simulink model "TP_Lab2_PI_TL081"  (R2026b)
settings: Solver=ode23t  StopTime=0.08  MaxStep=1e-5  RelTol=1e-6  AbsTol=1e-8
libraries: fl_lib x28, ee_lib x5, nesl_utility x3
settings Model: Creator=Usuario  LastModifiedBy=Usuario
settings SimscapeCC: SimscapeLogType=all  SimscapeNominalValues="[{\"value\":\"1\",\"unit\":\"A\"},{\"value\":\"1\",\"unit\":\"bar\"},{\"value\":\"1\",\"unit\":\"cm^2\"},{\"value\":\"1\",\"unit\":\"cm^3/s\"},{\"value\":\"1\",\"unit\":\"kJ/kg\"},{\"value\":\"1\",\"unit\":\"kW\"},{\"value\":\"1\",\"unit\":\"l\"},{\"value\":\"1\",\"unit\":\"N\"},{\"value\":\"1\",\"unit\":\"N*m\"},{\"value\":\"1\",\"unit\":\"V\"},{\"value\":\"0.001\",\"unit\":\"Wb\"}]"  SimscapeUseEnergyAccounting=off

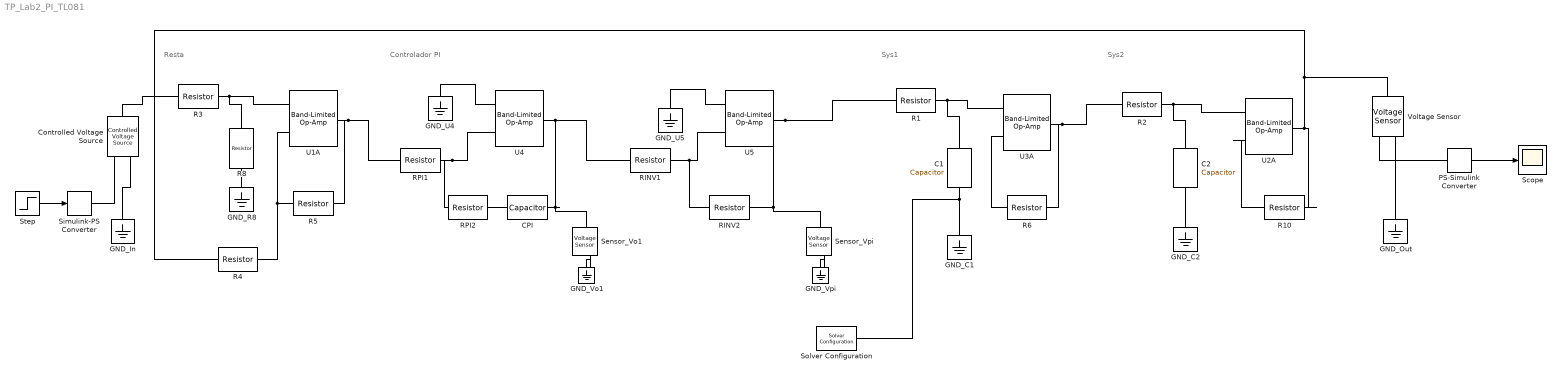
== system TP_Lab2_PI_TL081 ==
  note: Resta
  note: Sys1
  note: Sys2
  note: Controlador PI
  C1 : fl_lib/Electrical/Electrical Elements/Capacitor  c=0.1 uF  r=0 Ohm  g=0 1/Ohm  i_specify=off  i_priority=None  i=0 A  i_nominal_specify=off  i_nominal_value=1  i_nominal_unit=A  v_specify=off  v_priority=None  v=0 V  v_nominal_specify=off  v_nominal_value=1  v_nominal_unit=V  vc_specify=on  vc_priority=High  vc=0 V  vc_nominal_specify=off  vc_nominal_value=1  vc_nominal_unit=V
  C2 : fl_lib/Electrical/Electrical Elements/Capacitor  c=0.1 uF  r=0 Ohm  g=0 1/Ohm  i_specify=off  i_priority=None  i=0 A  i_nominal_specify=off  i_nominal_value=1  i_nominal_unit=A  v_specify=off  v_priority=None  v=0 V  v_nominal_specify=off  v_nominal_value=1  v_nominal_unit=V  vc_specify=on  vc_priority=High  vc=0 V  vc_nominal_specify=off  vc_nominal_value=1  vc_nominal_unit=V
  CPI : fl_lib/Electrical/Electrical Elements/Capacitor  c=0.1 uF  r=0 Ohm  g=0 1/Ohm  i_specify=off  i_priority=None  i=0 A  i_nominal_specify=off  i_nominal_value=1  i_nominal_unit=A  v_specify=off  v_priority=None  v=0 V  v_nominal_specify=off  v_nominal_value=1  v_nominal_unit=V  vc_specify=on  vc_priority=High  vc=0 V  vc_nominal_specify=off  vc_nominal_value=1  vc_nominal_unit=V
  Controlled Voltage Source : fl_lib/Electrical/Electrical Sources/Controlled Voltage Source
  GND_C1 : fl_lib/Electrical/Electrical Elements/Electrical Reference
  GND_C2 : fl_lib/Electrical/Electrical Elements/Electrical Reference
  GND_In : fl_lib/Electrical/Electrical Elements/Electrical Reference
  GND_Out : fl_lib/Electrical/Electrical Elements/Electrical Reference
  GND_R8 : fl_lib/Electrical/Electrical Elements/Electrical Reference
  GND_U4 : fl_lib/Electrical/Electrical Elements/Electrical Reference
  GND_U5 : fl_lib/Electrical/Electrical Elements/Electrical Reference
  GND_Vo1 : fl_lib/Electrical/Electrical Elements/Electrical Reference
  GND_Vpi : fl_lib/Electrical/Electrical Elements/Electrical Reference
  PS-Simulink Converter : nesl_utility/PS-Simulink Converter  PhysicalDomain=network_engine_domain  SubClassName=ps_output  LeftPortType=input  RightPortType=output  PseudoPeriodic=off  Frequencies=[]  VectorFormat=inherit  Unit=inherit  AffineConversion=off
  R1 : fl_lib/Electrical/Electrical Elements/Resistor  R=100 kOhm  i_specify=off  i_priority=None  i=0 A  i_nominal_specify=off  i_nominal_value=1  i_nominal_unit=A  v_specify=off  v_priority=None  v=0 V  v_nominal_specify=off  v_nominal_value=1  v_nominal_unit=V
  R{3..6,8,10} (6 alike) : fl_lib/Electrical/Electrical Elements/Resistor  R=1 kOhm  i_specify=off  i_priority=None  i=0 A  i_nominal_specify=off  i_nominal_value=1  i_nominal_unit=A  v_specify=off  v_priority=None  v=0 V  v_nominal_specify=off  v_nominal_value=1  v_nominal_unit=V
  R2 : fl_lib/Electrical/Electrical Elements/Resistor  R=47 kOhm  i_specify=off  i_priority=None  i=0 A  i_nominal_specify=off  i_nominal_value=1  i_nominal_unit=A  v_specify=off  v_priority=None  v=0 V  v_nominal_specify=off  v_nominal_value=1  v_nominal_unit=V
  RINV1 : fl_lib/Electrical/Electrical Elements/Resistor  R=10 kOhm  i_specify=off  i_priority=None  i=0 A  i_nominal_specify=off  i_nominal_value=1  i_nominal_unit=A  v_specify=off  v_priority=None  v=0 V  v_nominal_specify=off  v_nominal_value=1  v_nominal_unit=V
  RINV2 : fl_lib/Electrical/Electrical Elements/Resistor  R=10 kOhm  i_specify=off  i_priority=None  i=0 A  i_nominal_specify=off  i_nominal_value=1  i_nominal_unit=A  v_specify=off  v_priority=None  v=0 V  v_nominal_specify=off  v_nominal_value=1  v_nominal_unit=V
  RPI1 : fl_lib/Electrical/Electrical Elements/Resistor  R=120 kOhm  i_specify=off  i_priority=None  i=0 A  i_nominal_specify=off  i_nominal_value=1  i_nominal_unit=A  v_specify=off  v_priority=None  v=0 V  v_nominal_specify=off  v_nominal_value=1  v_nominal_unit=V
  RPI2 : fl_lib/Electrical/Electrical Elements/Resistor  R=82 kOhm  i_specify=off  i_priority=None  i=0 A  i_nominal_specify=off  i_nominal_value=1  i_nominal_unit=A  v_specify=off  v_priority=None  v=0 V  v_nominal_specify=off  v_nominal_value=1  v_nominal_unit=V
  Scope : Scope
  Sensor_Vo1 : fl_lib/Electrical/Electrical Sensors/Voltage Sensor
  Sensor_Vpi : fl_lib/Electrical/Electrical Sensors/Voltage Sensor
  Simulink-PS Converter : nesl_utility/Simulink-PS Converter  PhysicalDomain=network_engine_domain  SubClassName=ps_input  LeftPortType=input  RightPortType=output  PseudoPeriodic=off  Frequencies=[]  NoiseDistribution=none  NoiseParameters=[]  Unit=1  AffineConversion=off  FilteringAndDerivatives=provide  SimscapeFilterOrder=1  InputFilterTimeConstant=0.001  UdotUserProvided=0
  Solver Configuration : nesl_utility/Solver Configuration  PhysicalDomain=network_engine_domain  SubClassName=solver  LeftPortType=input  RightPortType=generic  Tones=[]  Harmonics=[]  SimulateNoise=off  Profile=off  UseLocalSampling=off  EnableSwitchedLinearOptims=on  FrequencyDomain=off  UseCCode=off  RelTol=0.001  AbsTol=0.001  MinStep=1e-09  ToWorkspace=off  RevertToSquareIcSolve=off  NumHomotopyIterations=100  PhasorMode=off  PhasorModeNumHarmonics=1  ConsistencySolver=NEWTON_XTOL_AFTER_FTOL  CanonicalOrdering=CANONICAL  OptimizeIntermediates=OPTIMIZED  MulticoreSolverChoice=BACKWARD_EULER  IndexReductionMethod=DerivativeReplacement  DoDC=off  ResidualTolerance=1e-09  ConsistencyTolSource=GLOBAL  ConsistencyAbsTol=0.001  ConsistencyRelTol=0.001  ConsistencyTolFactor=0.001  UseLocalSolver=off  LocalSolverChoice=NE_BACKWARD_EULER_ADVANCER  ResolveIndetEquations=on  FunctionEvalNumThread=1  LocalSolverSampleTime=0.001  DoFixedCost=off  MaxNonlinIter=3  MaxModeIter=2  ComputeImpulses=off  ImpulseIterations=2  LinearAlgebra=auto  LinearAlgebraNumThread=0  EquationFormulation=NE_TIME_EF  DelaysMemoryBudget=1024  AutomaticFiltering=on  FilteringTimeConstant=0.001  PartitionStorageMethod=AS_NEEDED  PartitionMemoryBudget=1024  PartitionMethod=BALANCED  MultibodyUseLocalSolver=off  MultibodyLocalSolverChoice=ODE1  MultibodyLocalSolverSampleTime=0.001
  Step : Step  Time=0  SampleTime=0
  U1A : ee_lib/Integrated Circuits/Band-Limited Op-Amp  A=2e5  Rin=1e12 Ohm  Rout=0 Ohm  Vmin=-8.5 V  Vmax=8.5 V  Vdotmax=13e6 V/s  f=15 Hz  V0=0 V
  U2A : ee_lib/Integrated Circuits/Band-Limited Op-Amp  A=2e5  Rin=1e12 Ohm  Rout=0 Ohm  Vmin=-8.5 V  Vmax=8.5 V  Vdotmax=13e6 V/s  f=15 Hz  V0=0 V
  U3A : ee_lib/Integrated Circuits/Band-Limited Op-Amp  A=2e5  Rin=1e12 Ohm  Rout=0 Ohm  Vmin=-8.5 V  Vmax=8.5 V  Vdotmax=13e6 V/s  f=15 Hz  V0=0 V
  U4 : ee_lib/Integrated Circuits/Band-Limited Op-Amp  A=2e5  Rin=1e12 Ohm  Rout=0 Ohm  Vmin=-8.5 V  Vmax=8.5 V  Vdotmax=13e6 V/s  f=15 Hz  V0=0 V
  U5 : ee_lib/Integrated Circuits/Band-Limited Op-Amp  A=2e5  Rin=1e12 Ohm  Rout=0 Ohm  Vmin=-8.5 V  Vmax=8.5 V  Vdotmax=13e6 V/s  f=15 Hz  V0=0 V
  Voltage Sensor : fl_lib/Electrical/Electrical Sensors/Voltage Sensor
  wires:
  Step/1 -> Simulink-PS Converter/1
  PS-Simulink Converter/1 -> Scope/1
  connections:
  Simulink-PS Converter/RConn1 -- Controlled Voltage Source/RConn1
  Controlled Voltage Source/RConn2 -- GND_In/LConn1
  Controlled Voltage Source/LConn1 -- R3/LConn1
  U1A/LConn1 -- R3/RConn1 -- R8/LConn1
  R8/RConn1 -- GND_R8/LConn1
  R5/LConn1 -- U1A/LConn2 -- R4/LConn1
  R5/RConn1 -- U1A/RConn1 -- RPI1/LConn1
  GND_U4/LConn1 -- U4/LConn1
  U4/LConn2 -- RPI1/RConn1 -- RPI2/LConn1
  RPI2/RConn1 -- CPI/LConn1
  CPI/RConn1 -- Sensor_Vo1/LConn1 -- U4/RConn1 -- RINV1/LConn1
  Sensor_Vo1/RConn2 -- GND_Vo1/LConn1
  GND_U5/LConn1 -- U5/LConn1
  U5/LConn2 -- RINV1/RConn1 -- RINV2/LConn1
  RINV2/RConn1 -- Sensor_Vpi/LConn1 -- U5/RConn1 -- R1/LConn1
  Sensor_Vpi/RConn2 -- GND_Vpi/LConn1
  U3A/LConn1 -- R1/RConn1 -- C1/LConn1
  GND_C1/LConn1 -- C1/RConn1 -- Solver Configuration/RConn1
  U3A/LConn2 -- R6/LConn1
  R6/RConn1 -- U3A/RConn1 -- R2/LConn1
  U2A/LConn1 -- R2/RConn1 -- C2/LConn1
  C2/RConn1 -- GND_C2/LConn1
  U2A/LConn2 -- R10/LConn1
  R10/RConn1 -- Voltage Sensor/LConn1 -- R4/RConn1 -- U2A/RConn1
  Voltage Sensor/RConn2 -- GND_Out/LConn1
  Voltage Sensor/RConn1 -- PS-Simulink Converter/LConn1
